simulink model "logic_flight"  (R2025b)
settings: Solver=VariableStepAuto  StartTime=0.0  StopTime=20  RelTol=1e-3
values from neighbouring files (symbols this model uses):
  A = zeros(12,12)    [Quadcoter.m]
  B = zeros(12,4)    [Quadcoter.m]
  C = zeros(4,12)    [Quadcoter.m]
  K = place(A,B,vp)    [Quadcoter.m]
  N = pinv(G0)    [Quadcoter.m]
  x0 = zeros(12,1)    [Quadcoter.m]
settings Model: Creator=user  LastModifiedBy=user

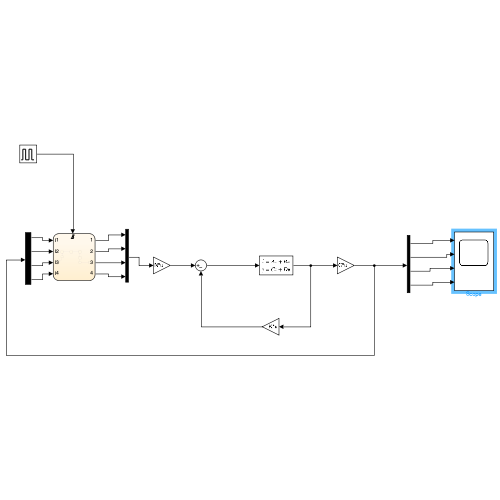
[thumbnail: Simulink's stored preview of the top-level diagram]
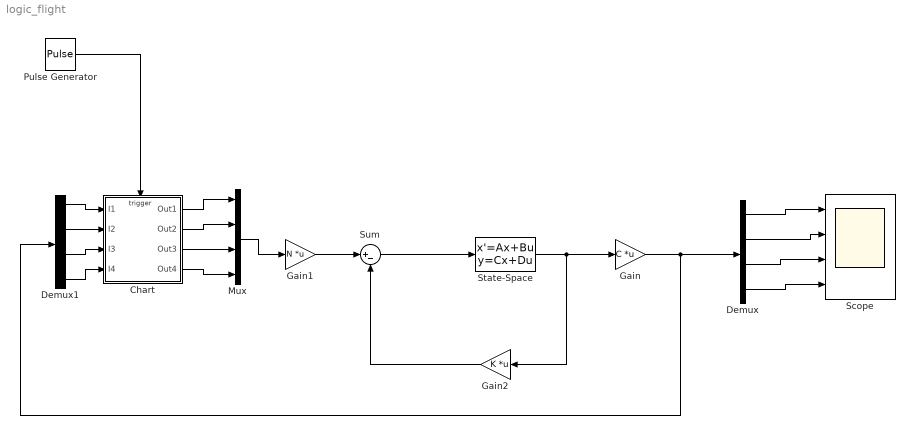
== system logic_flight ==
  Chart : Stateflow chart  TreatAsAtomicUnit=on
  Demux : Demux
  Demux1 : Demux
  Gain : Gain  Gain=C  Multiplication=Matrix(K*u)
  Gain1 : Gain  Gain=N  Multiplication=Matrix(K*u)
  Gain2 : Gain  Gain=K  Multiplication=Matrix(K*u)
  Mux : Mux
  Pulse Generator : DiscretePulseGenerator  PulseType=Time based  Period=1  PulseWidth=50
  Scope : Scope  NumInputPorts=4
      settings: ActiveDisplayYMinimum=-1.9296758681974322  ActiveDisplayYMaximum=3.8632451427576311
  State-Space : StateSpace  A=A  B=B  C=eye(12,12)  D=zeros(12,4)  InitialCondition=x0
  Sum : Sum  Inputs=|+-
  wires:
  Sum/1 -> State-Space/1
  State-Space/1 -> Gain2/1, Gain/1
  Demux/3 -> Scope/3
  Gain/1 -> Demux1/1, Demux/1
  Demux/4 -> Scope/4
  Demux/1 -> Scope/1
  Gain2/1 -> Sum/2
  Gain1/1 -> Sum/1
  Demux/2 -> Scope/2
  Chart/1(Out1) -> Mux/1
  Chart/2(Out2) -> Mux/2
  Chart/3(Out3) -> Mux/3
  Chart/4(Out4) -> Mux/4
  Mux/1 -> Gain1/1
  Pulse Generator/1 -> Chart/Trigger
  Demux1/1 -> Chart/1(I1)
  Demux1/2 -> Chart/2(I2)
  Demux1/3 -> Chart/3(I3)
  Demux1/4 -> Chart/4(I4)

== stateflow chart logic_flight/Chart ==
  state Hover_1
  state Cruise
    during:
    Out1 = In1,
    Out2 = In2;
  state Hover_arr
  state Lift
    entry:
    Out1 = In1,
    Out2 = In2,
    Out3 = In3,
    Out4 = In4;
  state Descend_1
    entry:
    Out1 = In1,
    Out2 = In2,
    Out3 = In3;
  state Start
    entry:
    In1 = 0,
    In2 = 0,
    In3 = 0,
    In4 = 0;
  state Lift1
    entry:
    Out1 = In1,
    Out2 = In2,
    Out3 = In3;
  state Hover_drop
  Hover_1 -> Cruise : [after(3, sec)]{In1=2; In2=3}
  Cruise -> Hover_arr : [I1>=2 && I2 >=3]
  Hover_arr -> Descend_1 : [after(2, sec)]{In1=2; In2=3; In3=1.5}
  Lift -> Hover_1 : [I3 >=2]
  Start -> Lift : Start/{In1=0; In2=0; In3=2; In4=0}
  Descend_1 -> Hover_drop : [I3 <=1.6]
  (default) -> Start
  Hover_drop -> Lift1 : [after(2, sec)]{In1=2; In2=3; In3=2}
  data: Out1 output; Out2 output; Out3 output; Out4 output; In1 local; In2 local; In3 local; In4 local; I1 input; I2 input; I3 input; I4 input
  events: Start input RISING_EDGE_EVENT
